simulink model "P2_E"  (R2024b)
settings: Solver=VariableStepAuto  StartTime=0.0  StopTime=10.0  RelTol=1e-3
settings Model: Creator=sepeh  LastModifiedBy=sepeh

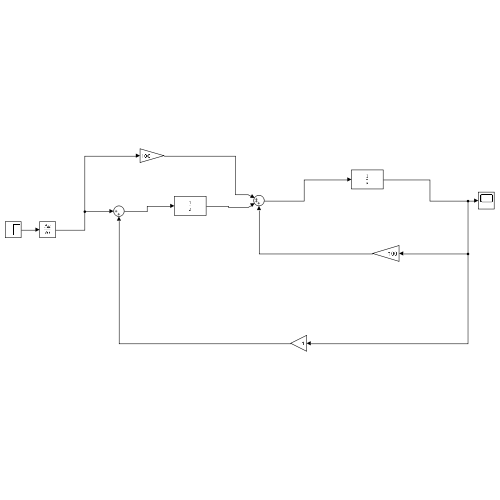
[thumbnail: Simulink's stored preview of the top-level diagram]
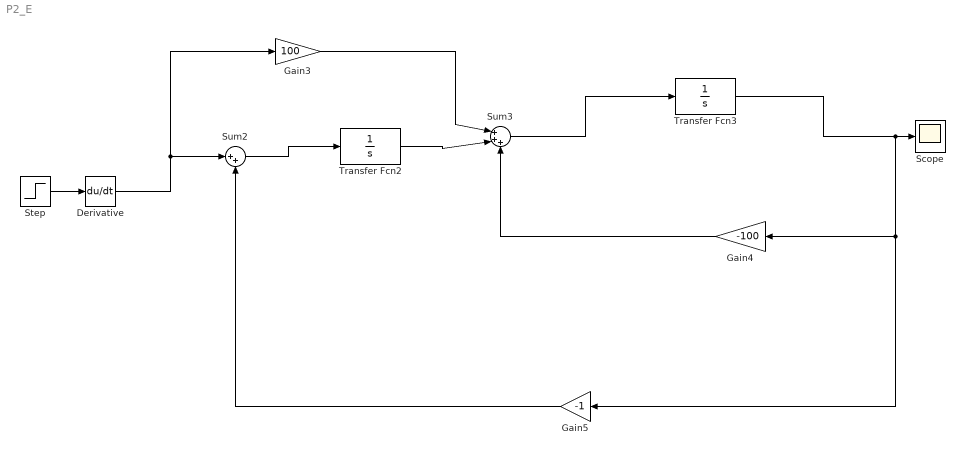
== system P2_E ==
  Derivative : Derivative
  Gain3 : Gain  Gain=100
  Gain4 : Gain  Gain=-100
  Gain5 : Gain  Gain=-1
  Scope : Scope
  Step : Step  Time=0.000001  SampleTime=0
  Sum2 : Sum  Inputs=|++
  Sum3 : Sum  Inputs=|+++
  Transfer Fcn2 : TransferFcn  Denominator="[1  0]"
  Transfer Fcn3 : TransferFcn  Denominator="[1  0]"
  wires:
  Step/1 -> Derivative/1
  Transfer Fcn3/1 -> Gain5/1, Gain4/1, Scope/1
  Derivative/1 -> Gain3/1, Sum2/1
  Sum2/1 -> Transfer Fcn2/1
  Transfer Fcn2/1 -> Sum3/2
  Gain4/1 -> Sum3/3
  Gain3/1 -> Sum3/1
  Gain5/1 -> Sum2/2
  Sum3/1 -> Transfer Fcn3/1
